simulink model "au50_hbm_data_test"  (R2021a)
settings: Solver=VariableStepDiscrete  StartTime=0.0  StopTime=3000  RelTol=1e-3
libraries: xbsIndex_r4 x618, casper_library_misc x3, xps_library x2
(part 4 of 10)

== system au50_hbm_data_test/hbm_in_rd_snap/ss/bram ==
  addr : Inport
  data_in : Inport  Port=2
  we : Inport  Port=3
  Terminator : Terminator
  Terminator1 : Terminator
  Terminator2 : Terminator
  au50_hbm_data_test_hbm_in_rd_snap_ss_bram_addr : xbsIndex_r4/Gateway Out  inherit_from_input=off  hdl_port=on  rows=1  columns=1  UseAsDAC=off  DACChannel='1'  interface=None  automatic_assignment=on  address_offset=hex2dec('00')  intf_name=''  intf_description=''  timing_constraint=None  locs_specified=off  LOCs={'A5','B9','A9','C1','A3','G6','E9','A6','A7','A8','B8','B1','B3','D9','B5','B4','B6','C2'}  io_standard={}  block_type=gatewayout
      settings: infoedit="Gateway out block.  Converts Xilinx fixed point inputs into ouputs of type Simulink integer, double, or fixed point.<P><P>Hardware notes:  In hardware these blocks become top level output ports or are discarded, depending on how they are configured."  sginterface={'Nallatech'=>{'xdspkit'=>{'non_memory_mapped_port'=>'uprev_Shared_BRAM_addr'}},'Xilinx'=>{'jtaghwcosim'=>{'non_memory_mapped_port'=>'uprev_Shared_BRAM_addr'},'xdspkit'=>{'non_memory_mapped_port'=>'uprev_Shared_BRAM_addr'}}}  xl_area=[0, 0, 0, 0, 0, 0, 0]
  au50_hbm_data_test_hbm_in_rd_snap_ss_bram_data_in : xbsIndex_r4/Gateway Out  inherit_from_input=off  hdl_port=on  rows=1  columns=1  UseAsDAC=off  DACChannel='1'  interface=None  automatic_assignment=on  address_offset=hex2dec('00')  intf_name=''  intf_description=''  timing_constraint=None  locs_specified=off  LOCs={'B21','B22','A22','B23','B19','C19','A20','A21','A23','B24','A24','A25','E18','D18','C18','B18'}  io_standard={}  block_type=gatewayout
      settings: infoedit="Gateway out block.  Converts Xilinx fixed point inputs into ouputs of type Simulink integer, double, or fixed point.<P><P>Hardware notes:  In hardware these blocks become top level output ports or are discarded, depending on how they are configured."  sginterface={'Nallatech'=>{'xdspkit'=>{'non_memory_mapped_port'=>'uprev_Shared_BRAM_data_in'}},'Xilinx'=>{'jtaghwcosim'=>{'non_memory_mapped_port'=>'uprev_Shared_BRAM_data_in'},'xdspkit'=>{'non_memory_mapped_port'=>'uprev_Shared_BRAM_data_in'}}}  xl_area=[0, 0, 0, 0, 0, 0, 0]
  au50_hbm_data_test_hbm_in_rd_snap_ss_bram_data_out : xbsIndex_r4/Gateway In  gui_display_data_type=Fixed-point  arith_type=Unsigned  n_bits=64  bin_pt=0  preci_type=Single  exp_width=8  frac_width=24  rows=1  columns=1  quantization=Truncate  overflow=Wrap  period=sample_rate  UseAsADC=off  ADCChannel='1'  interface=None  automatic_assignment=on  address_offset=hex2dec('00')  intf_name=''  intf_description=''  default_value=0  timing_constraint=None  locs_specified=off  LOCs={}  io_standard={}  inherit_from_input=off  hdl_port=on  dbl_ovrd=off  block_type=gatewayin
      settings: xl_area=[0, 0, 0, 0, 0, 0, 0]
  au50_hbm_data_test_hbm_in_rd_snap_ss_bram_we : xbsIndex_r4/Gateway Out  inherit_from_input=off  hdl_port=on  rows=1  columns=1  UseAsDAC=off  DACChannel='1'  interface=None  automatic_assignment=on  address_offset=hex2dec('00')  intf_name=''  intf_description=''  timing_constraint=None  locs_specified=off  LOCs={'A14'}  io_standard={}  block_type=gatewayout
      settings: infoedit="Gateway out block.  Converts Xilinx fixed point inputs into ouputs of type Simulink integer, double, or fixed point.<P><P>Hardware notes:  In hardware these blocks become top level output ports or are discarded, depending on how they are configured."  xl_area=[0, 0, 0, 0, 0, 0, 0]
  calc_add : Subsystem  mask{data_width=64, addr_width=13, sample_rate=sample_rate}
      mask prompts: data_width "data width"; addr_width "address width"; sample_rate "sample rate"
  convert_addr : xbsIndex_r4/Convert  gui_display_data_type=Fixed-point  arith_type=Unsigned  n_bits=addr_width  bin_pt=0  float_type=Single  exp_bits=8  fraction_bits=24  quantization=Truncate  overflow=Wrap  en=off  latency=0  pipeline=off  dbl_ovrd=off  block_type=convert
      settings: xl_area=[0, 0, 0, 0, 0, 0, 0]
  convert_din1 : xbsIndex_r4/Convert  gui_display_data_type=Fixed-point  arith_type=Unsigned  n_bits=64  bin_pt=0  float_type=Single  exp_bits=8  fraction_bits=24  quantization=Truncate  overflow=Wrap  en=off  latency=0  pipeline=off  dbl_ovrd=off  block_type=convert
      settings: xl_area=[0, 0, 0, 0, 0, 0, 0]
  convert_we : xbsIndex_r4/Convert  gui_display_data_type=Fixed-point  arith_type=Unsigned  n_bits=1  bin_pt=0  float_type=Single  exp_bits=8  fraction_bits=24  quantization=Truncate  overflow=Wrap  en=off  latency=0  pipeline=off  dbl_ovrd=off  block_type=convert
      settings: xl_area=[0, 0, 0, 0, 0, 0, 0]
  munge_in : Subsystem  AncestorBlock=casper_library_flow_control/munge  mask(munge){divisions=2, div_size=[32 32], order=[1  0], arith_type_out=Unsigned, bin_pt_out=0}
      mask prompts: divisions "Number of divisions"; div_size "Division size (bits)"; order "Division packing order"; arith_type_out "Output arithmetic type"; bin_pt_out "Output binary point"
      mask help: Splits an input bus into the specified number of divisions and then recombines them in the order specified (most significant division = 0,least = number divisions-1)
      mask init:
      | munge_init(gcb, ...
      |     'divisions', divisions, ...
      |     'div_size', div_size, ...
      |     'order', order, ...
      |     'arith_type_out', arith_type_out, ...
      |     'bin_pt_out', bin_pt_out);
      settings: AttributesFormatString=|
      | split:[32 32]
      | join:[1 0]
      | Unsigned [64,0]
      mask TypeOptions arith_type_out: Unsigned | Signed  (2's comp) | Floating-point
  munge_out : Subsystem  AncestorBlock=casper_library_flow_control/munge  mask(munge){divisions=2, div_size=[32 32], order=[1  0], arith_type_out=Unsigned, bin_pt_out=0}
      mask prompts: divisions "Number of divisions"; div_size "Division size (bits)"; order "Division packing order"; arith_type_out "Output arithmetic type"; bin_pt_out "Output binary point"
      mask help: Splits an input bus into the specified number of divisions and then recombines them in the order specified (most significant division = 0,least = number divisions-1)
      mask init:
      | munge_init(gcb, ...
      |     'divisions', divisions, ...
      |     'div_size', div_size, ...
      |     'order', order, ...
      |     'arith_type_out', arith_type_out, ...
      |     'bin_pt_out', bin_pt_out);
      settings: AttributesFormatString=|
      | split:[32 32]
      | join:[1 0]
      | Unsigned [64,0]
      mask TypeOptions arith_type_out: Unsigned | Signed  (2's comp) | Floating-point
  sim_mem : Subsystem  mask{arith_type=Unsigned, addr_width=13, data_width=64, data_bin_pt=0, init_vals=[0     1     2     3     4     5     6     7     8     9    10    11    12    13    14    15    16    17    18    19    20    21    22    23    24    25    26    27    28    29    30    31    32    33    34    35    36    37    38    39    40    41    42    43    44    45    46    47    48    49    50    51    52    53    54    55    56    57    58    59    60    61    62    63    64    65    66    67    68    69    70    71    72    73    74    75    76    77    78    79    80    81    82    83    84    85    86    87    88    89    90    91    92    93    94    95    96    97    98    99   100   101   102   103   104   105   106   107   108   109   110   111   112   113   114   115   116   117   118   119   120   121   122   123   124   125   126   127   128   129   130   131   132   133   134   135   136   137   138   139   140   141   142   143   144   145   146   147   148   149   150   151   152   153   154   155   156   157   158   159   160   161   162   163   164   165   166   167   168   169   170   171   172   173   174   175   176   177   178   179   180   181   182   183   184   185   186   187   188   189   190   191   192   193   194   195   196   197   198   199   200   201   202   203   204   205   206   207   208   209   210   211   212   213   214   215   216   217   218   219   220   221   222   223   224   225   226   227   228   229   230   231   232   233   234   235   236   237   238   239   240   241   242   243   244   245   246   247   248   249   250   251   252   253   254   255   256   257   258   259   260   261   262   263   264   265   266   267   268   269   270   271   272   273   274   275   276   277   278   279   280   281   282   283   284   285   286   287   288   289   290   291   292   293   294   295   296   297   298   299   300   301   302   303   304   305   306   307   308   309   310   311   312   313   314   315   316   317   318   319   320   321   322   323   324   325   326   327   328   329   330   331   332   333   334   335   336   337   338   339   340   341   342   343   344   345   346   347   348   349   350   351   352   353   354   355   356   357   358   359   360   361   362   363   364   365   366   367   368   369   370   371   372   373   374   375   376   377   378   379   380   381   382   383   384   385   386   387   388   389   390   391   392   393   394   395   396   397   398   399   400   401   402   403   404   405   406   407   408   409   410   411   412   413   414   415   416   417   418   419   420   421   422   423   424   425   426   427   428   429   430   431   432   433   434   435   436   437   438   439   440   441   442   443   444   445   446   447   448   449   450   451   452   453   454   455   456   457   458   459   460   461   462   463   464   465   466   467   468   469   470   471   472   473   474   475   476   477   478   479   480   481   482   483   484   485   486   487   488   489   490   491   492   493   494   495   496   497   498   499   500   501   502   503   504   505   506   507   508   509   510   511   512   513   514   515   516   517   518   519   520   521   522   523   524   525   526   527   528   529   530   531   532   533   534   535   536   537   538   539   540   541   542   543   544   545   546   547   548   549   550   551   552   553   554   555   556   557   558   559   560   561   562   563   564   565   566   567   568   569   570   571   572   573   574   575   576   577   578   579   580   581   582   583   584   585   586   587   588   589   590   591   592   593   594   595   596   597   598   599   600   601   602   603   604   605   606   607   608   609   610   611   612   613   614   615   616   617   618   619   620   621   622   623   624   625   626   627   628   629   630   631   632   633   634   635   636   637   638   639   640   641   642   643   644   645   646   647   648   649   650   651   652   653   654   655   656   657   658   659   660   661   662   663   664   665   666 ...(+45149 chars)], sample_rate=1, csp_latency=1}
      mask prompts: arith_type "Output Data Type"; addr_width "Address width"; data_width "Data width"; data_bin_pt "Data Binary Point"; init_vals "Initial values"; sample_rate "Sample rate"; csp_latency "Latency"
      mask init:
      | % set_param([gcb, '/data_to_xilinx'], 'arith_type', arith_type)
      | % set_param([gcb, '/data_to_xilinx'], 'n_bits', get_param(gcb, 'data_width'))
      mask TypeOptions arith_type: Unsigned | Signed  (2's comp)
      mask TypeOptions data_width: 8 | 16 | 32 | 64 | 128
  data_out : Outport  VectorParamsAs1DForOutWhenUnconnected=off
  wires:
  munge_out/1(dout) -> data_out/1
  sim_mem/1(data_out) -> au50_hbm_data_test_hbm_in_rd_snap_ss_bram_data_out/1
  au50_hbm_data_test_hbm_in_rd_snap_ss_bram_data_out/1 -> munge_out/1(din)
  convert_addr/1 -> au50_hbm_data_test_hbm_in_rd_snap_ss_bram_addr/1
  convert_din1/1 -> au50_hbm_data_test_hbm_in_rd_snap_ss_bram_data_in/1
  data_in/1 -> munge_in/1(din)
  calc_add/1(out) -> sim_mem/1(addr), convert_addr/1
  au50_hbm_data_test_hbm_in_rd_snap_ss_bram_we/1 -> Terminator2/1
  au50_hbm_data_test_hbm_in_rd_snap_ss_bram_data_in/1 -> Terminator1/1
  au50_hbm_data_test_hbm_in_rd_snap_ss_bram_addr/1 -> Terminator/1
  convert_we/1 -> au50_hbm_data_test_hbm_in_rd_snap_ss_bram_we/1
  addr/1 -> calc_add/1(in)
  we/1 -> sim_mem/3(we), convert_we/1
  munge_in/1(dout) -> sim_mem/2(data), convert_din1/1
